simulink model "XFLUID02_reference"  (R2025a)
settings: Solver=ode23t  StartTime=0  StopTime=1.5  MaxStep=0.001  RelTol=1e-3  EnableMultiTasking=on
model workspace (MAT data in the model file):
  TRP_Par : object (value not decoded)
  fault_cylinder = 2
  inlet_area_factor = 1
  output_pressure_bar = 7
  pOutMeas_data = [7; 7]
  pOutMeas_time = [0; 1.5]
  pOut_Init_WKSP = 7
  pump_speed_rpm = 958
  seal_leak_fraction = 0
  speed_step_fraction = 0.08
  speed_step_time = 0.72
symbols that are objects in the model workspace (value not decoded): TRP_Par
undefined symbols (not defined in the file): Plunger, sm_pump_triplex_lib, smiData, X, Y, Z
libraries: sm_lib x133, fl_lib x62, nesl_utility x24, SimscapeFluids_lib x15, simulink x10, ee_lib x2
(part 7 of 7)

== system XFLUID02_reference/Pump/Plunger 3/Seal Leak/Tune ==
  Fixed Orifice : SimscapeFluids_lib/Isothermal Liquid/Valves & Orifices/Orifices/Orifice (IL)  orifice_type=1  constant_orifice_spec=fluids.isothermal_liquid.valves_orifices.orifices.enum.constant_orifice_spec.area  variable_orifice_spec=fluids.isothermal_liquid.valves_orifices.orifices.enum.orifice_spec.linear  orifice_area_constant=leak_cyl_area_WKSP m^2  p_diff_TLU_constant=[-4, -3, -2, -1, -.5, 0, .5, 1, 2, 3, 4] MPa  vol_flow_TLU_constant=[-2.44, -2.12, -1.68, -1.22, -.84, 0, .85, 1.21, 1.7, 2.09, 2.41] .* 1e-3 m^3/s  S_min=0 m  del_S=5e-3 m  open_orientation=fluids.isothermal_liquid.valves_orifices.orifices.enum.orifice_orientation.positive  area_max=1e-4 m^2  area_leak=1e-10 m^2  S_TLU=[0, .002, .004, .007, .017] m  orifice_area_TLU=[1e-09, 2.0352e-07, 4.0736e-05, .00011438, .00034356] m^2  area=inf m^2  Cd=0.7  Re_c=150  smoothing_factor=0.01  pressure_recovery=false  S_vol_flow_TLU=[0, .002, .004, .007, .017] m  p_diff_TLU=[.3, .5, .7] MPa  vol_flow_TLU=1e-3 * [1.7e-05, 2e-05, 2.6e-05; .0035, .0045, .0053; .7, .9, 1.06; 1.96, 2.5, 3; 6, 7.7, 9.13] m^3/s
      settings: LibrarySourceBlock=sh_lib/Orifices/Fixed Orifice  InternalSimscapePortConfiguration="{\"Bottom\":[],\"Left\":[{\"id\":\"A\",\"label\":\"A\",\"type\":\"foundation.isothermal_liquid.isothermal_liquid\"}],\"Right\":[{\"id\":\"B\",\"label\":\"B\",\"type\":\"foundation.isothermal_liquid.isothermal_liquid\"}],\"Top\":[]}"
  Hydraulic Reference : fl_lib/Isothermal Liquid/Elements/Reservoir (IL)  reservoir_type=foundation.enum.constant_controlled.constant  pressure_spec=foundation.enum.pressure_spec.atmospheric  reservoir_pressure=0.101325 MPa
      settings: LibrarySourceBlock=fl_lib/Hydraulic/Hydraulic Elements/Hydraulic Reference
  A : PMIOPort  Side=Left
  connections:
  Fixed Orifice/RConn1 -- Hydraulic Reference/LConn1
  Fixed Orifice/LConn1 -- A/RConn1

== system XFLUID02_reference/Pump/Plunger 3/Valve Visual/Off ==
  qi : Inport
  qo : Inport  Port=2
  Reference Frame : sm_lib/Frames and Transforms/Reference Frame
  Terminator : Terminator
  Terminator1 : Terminator
  W : PMIOPort  Side=Right
  wires:
  qi/1 -> Terminator1/1
  qo/1 -> Terminator/1
  connections:
  Reference Frame/RConn1 -- W/RConn1

== system XFLUID02_reference/Pump/Plunger 3/Valve Visual/On ==
  qi : Inport
  qo : Inport  Port=2
  Check Ball In : sm_lib/Body Elements/Spherical Solid  SphereRadius=chkv_vis_rad_in  SphereRadiusUnits=m  ExportEntireGeometry=off  InertiaType=CalculateFromGeometry  BasedOnType=Density  Density=1000  DensityUnits=kg/m^3  Mass=1  MassUnits=kg  CenterOfMass=[0 0 0]  CenterOfMassUnits=m  MomentsOfInertia=[1 1 1]  MomentsOfInertiaUnits=kg*m^2  ProductsOfInertia=[1 1 1]  ProductsOfInertiaUnits=kg*m^2  GraphicType=FromGeometry  MarkerShape=Sphere  MarkerSize=10  GraphicVisPropType=SimpleVisualProperties  GraphicDiffuseColor=chkv_vis_clr_in  GraphicOpacity=1.0  GraphicSpecularColor=[0.5 0.5 0.5 1.0]  GraphicAmbientColor=[0.15 0.15 0.15 1.0]  GraphicEmissiveColor=[0.0 0.0 0.0 1.0]  GraphicShininess=75  DoExposeReferenceFrame=on  SerializedFrames=<Frames/>
  Check Ball Out : sm_lib/Body Elements/Spherical Solid  SphereRadius=chkv_vis_rad_out  SphereRadiusUnits=m  ExportEntireGeometry=off  InertiaType=CalculateFromGeometry  BasedOnType=Density  Density=1000  DensityUnits=kg/m^3  Mass=1  MassUnits=kg  CenterOfMass=[0 0 0]  CenterOfMassUnits=m  MomentsOfInertia=[1 1 1]  MomentsOfInertiaUnits=kg*m^2  ProductsOfInertia=[1 1 1]  ProductsOfInertiaUnits=kg*m^2  GraphicType=FromGeometry  MarkerShape=Sphere  MarkerSize=10  GraphicVisPropType=SimpleVisualProperties  GraphicDiffuseColor=chkv_vis_clr_out  GraphicOpacity=1.0  GraphicSpecularColor=[0.5 0.5 0.5 1.0]  GraphicAmbientColor=[0.15 0.15 0.15 1.0]  GraphicEmissiveColor=[0.0 0.0 0.0 1.0]  GraphicShininess=75  DoExposeReferenceFrame=on  SerializedFrames=<Frames/>
  Gain : Gain  Gain=-1
  Prismatic Check Ball In : sm_lib/Joints/Prismatic Joint  JointMode=Normal  CompositeWrenchDir=FollowerOnBase  CompositeWrenchFrame=BaseFrame  SenseConstraintForce=off  SenseConstraintTorque=off  SenseTotalForce=off  SenseTotalTorque=off  PositionTargetSpecify=off  PositionTargetPriority=High  PositionTargetValue=0  PositionTargetValueUnits=m  VelocityTargetSpecify=off  VelocityTargetPriority=High  VelocityTargetValue=0  VelocityTargetValueUnits=m/s  EquilibriumPosition=0  EquilibriumPositionUnits=m  SpringStiffness=0  SpringStiffnessUnits=N/m  DampingCoefficient=0  DampingCoefficientUnits=N/(m/s)  LowerLimitSpecify=off  LowerLimitBound=-1  LowerLimitBoundUnits=m  LowerLimitStiffness=1e6  LowerLimitStiffnessUnits=N/m  LowerLimitDamping=1e3  LowerLimitDampingUnits=N/(m/s)  LowerLimitTransitionRegionWidth=1e-4  LowerLimitTransitionRegionWidthUnits=m  UpperLimitSpecify=off  UpperLimitBound=1  UpperLimitBoundUnits=m  UpperLimitStiffness=1e6  UpperLimitStiffnessUnits=N/m  UpperLimitDamping=1e3  UpperLimitDampingUnits=N/(m/s)  UpperLimitTransitionRegionWidth=1e-4  UpperLimitTransitionRegionWidthUnits=m  TorqueActuationMode=ComputedTorque  MotionActuationMode=InputMotion  SensePosition=off  SenseVelocity=off  SenseAcceleration=off  SenseTorqueForce=off  SenseLowerLimitTorqueForce=off  SenseUpperLimitTorqueForce=off
  Prismatic Check Ball Out : sm_lib/Joints/Prismatic Joint  JointMode=Normal  CompositeWrenchDir=FollowerOnBase  CompositeWrenchFrame=BaseFrame  SenseConstraintForce=off  SenseConstraintTorque=off  SenseTotalForce=off  SenseTotalTorque=off  PositionTargetSpecify=off  PositionTargetPriority=High  PositionTargetValue=0  PositionTargetValueUnits=m  VelocityTargetSpecify=off  VelocityTargetPriority=High  VelocityTargetValue=0  VelocityTargetValueUnits=m/s  EquilibriumPosition=0  EquilibriumPositionUnits=m  SpringStiffness=0  SpringStiffnessUnits=N/m  DampingCoefficient=0  DampingCoefficientUnits=N/(m/s)  LowerLimitSpecify=off  LowerLimitBound=-1  LowerLimitBoundUnits=m  LowerLimitStiffness=1e6  LowerLimitStiffnessUnits=N/m  LowerLimitDamping=1e3  LowerLimitDampingUnits=N/(m/s)  LowerLimitTransitionRegionWidth=1e-4  LowerLimitTransitionRegionWidthUnits=m  UpperLimitSpecify=off  UpperLimitBound=1  UpperLimitBoundUnits=m  UpperLimitStiffness=1e6  UpperLimitStiffnessUnits=N/m  UpperLimitDamping=1e3  UpperLimitDampingUnits=N/(m/s)  UpperLimitTransitionRegionWidth=1e-4  UpperLimitTransitionRegionWidthUnits=m  TorqueActuationMode=ComputedTorque  MotionActuationMode=InputMotion  SensePosition=off  SenseVelocity=off  SenseAcceleration=off  SenseTorqueForce=off  SenseLowerLimitTorqueForce=off  SenseUpperLimitTorqueForce=off
  Simulink-PS Converter : nesl_utility/Simulink-PS Converter  PhysicalDomain=network_engine_domain  SubClassName=ps_input  LeftPortType=input  RightPortType=output  PseudoPeriodic=off  Frequencies=[]  NoiseDistribution=none  NoiseParameters=[]  Unit=m  AffineConversion=off  FilteringAndDerivatives=filter  SimscapeFilterOrder=2  InputFilterTimeConstant=0.005  UdotUserProvided=0
  Simulink-PS Converter1 : nesl_utility/Simulink-PS Converter  PhysicalDomain=network_engine_domain  SubClassName=ps_input  LeftPortType=input  RightPortType=output  PseudoPeriodic=off  Frequencies=[]  NoiseDistribution=none  NoiseParameters=[]  Unit=m  AffineConversion=off  FilteringAndDerivatives=filter  SimscapeFilterOrder=2  InputFilterTimeConstant=0.005  UdotUserProvided=0
  Transform Inlet : sm_lib/Frames and Transforms/Rigid Transform  RotationMethod=None  FollAlignAxisA=+X  BaseAlignAxisA=+Y  FollAlignAxisB=+Y  BaseAlignAxisB=+Z  RotationStandardAxis=+Z  RotationAngle=0.0  RotationAngleUnits=deg  RotationArbitraryAxis=[0 0 1]  RotationSequenceAxes=FollowerAxes  RotationSequence=XYX  RotationSequenceAngles=[0 0 0]  RotationSequenceAnglesUnits=deg  RotationMatrix=[1 0 0; 0 1 0; 0 0 1]  Quaternion=[1 0 0 0]  TranslationMethod=Cartesian  TranslationCartesianOffset=[0 -0.04 -0.055-0.005]  TranslationCartesianOffsetUnits=m  TranslationStandardAxis=+Z  TranslationStandardOffset=0  TranslationStandardOffsetUnits=m  TranslationROffset=0  TranslationROffsetUnits=m  TranslationThetaOffset=0  TranslationThetaOffsetUnits=deg  TranslationZOffset=0  TranslationZOffsetUnits=m
  Transform Outlet : sm_lib/Frames and Transforms/Rigid Transform  RotationMethod=StandardAxis  FollAlignAxisA=+X  BaseAlignAxisA=+Y  FollAlignAxisB=+Y  BaseAlignAxisB=+Z  RotationStandardAxis=-X  RotationAngle=90  RotationAngleUnits=deg  RotationArbitraryAxis=[0 0 1]  RotationSequenceAxes=FollowerAxes  RotationSequence=XYX  RotationSequenceAngles=[0 0 0]  RotationSequenceAnglesUnits=deg  RotationMatrix=[1 0 0; 0 1 0; 0 0 1]  Quaternion=[1 0 0 0]  TranslationMethod=Cartesian  TranslationCartesianOffset=[0 0.020 -0.063]  TranslationCartesianOffsetUnits=m  TranslationStandardAxis=+Z  TranslationStandardOffset=0  TranslationStandardOffsetUnits=m  TranslationROffset=0  TranslationROffsetUnits=m  TranslationThetaOffset=0  TranslationThetaOffsetUnits=deg  TranslationZOffset=0  TranslationZOffsetUnits=m
  W : PMIOPort  Side=Right
  wires:
  Gain/1 -> Simulink-PS Converter/1
  qo/1 -> Simulink-PS Converter1/1
  qi/1 -> Gain/1
  connections:
  Simulink-PS Converter1/RConn1 -- Prismatic Check Ball Out/LConn2
  Prismatic Check Ball Out/RConn1 -- Check Ball Out/RConn1
  Prismatic Check Ball Out/LConn1 -- Transform Outlet/RConn1
  Simulink-PS Converter/RConn1 -- Prismatic Check Ball In/LConn2
  Transform Inlet/RConn1 -- Prismatic Check Ball In/LConn1
  W/RConn1 -- Transform Inlet/LConn1 -- Transform Outlet/LConn1
  Prismatic Check Ball In/RConn1 -- Check Ball In/RConn1

== system XFLUID02_reference/Driver/Driver/Motor/Windings/Enable if rotor angle 0-240 Deg ==
  Ang : Inport
  Constant2 : Constant  Value=360
  Interval Test : simulink/Logic and Bit Operations/Interval Test  IntervalClosedRight=on  uplimit=240  IntervalClosedLeft=on  lowlimit=0  OutDataTypeStr=uint8
      settings: AttributesFormatString=%<lowlimit><angle<%<uplimit>
  Math Function : Math  Operator=rem  SignedPower=on
  En : Outport  VectorParamsAs1DForOutWhenUnconnected=off
  wires:
  Constant2/1 -> Math Function/2
  Math Function/1 -> Interval Test/1
  Interval Test/1 -> En/1
  Ang/1 -> Math Function/1

== matlab function XFLUID02_reference/Diagnostics/Diagnostics/On/FFT and Classification ==
  data: pArray input; faultState output; enablePred input; cmdSpeed input; hmiVec output
function [faultState,hmiVec] = faultClassifier(pArray,enablePred,cmdSpeed)

% Initialize Predicted Machine State
faultState = int8(0);
hmiVec = [1 0 0 0];

% Sampling Parameters
Np = 1000;
Dt = 0.001;
numFreqPeaks = 5;

% Initialize Prediction Algorithm Input
predIn = NaN(1,2*numFreqPeaks+1);

pAvg = mean(pArray);

% Load Trained Machine Learning Algorithm
pumpPredict = loadLearnerForCoder('sm_pump_triplex_fault_detect_algo');

if enablePred
    
    % Compute FFT of Accumulated Data
    [freq,mag] = getFFTData(Np,pArray,Dt);
    
    % Normalize FFT Results
    freqFaultSpd = freq*60/(2*pi)/(cmdSpeed*3);

    % Detect FFT Peak Frequencies
    [pks,loc] = findpeaks(mag,'MinPeakProminence',0.5e-3);

    % Center FFT Peak Frequencies around Primary Machine Frequency
    normSpd = abs(freqFaultSpd(loc)-1);
    [sortFreq,sortIdx] = sort(normSpd);
    sortMag = pks(sortIdx);

    % Only Update Detected Peaks
    if length(sortMag) <= numFreqPeaks
        numFreq = length(sortMag);
    else
        numFreq = numFreqPeaks;
    end
    
    % Construct Input Array for Machine Learning Algorithm
    for i = 1:numFreq
        predIn(2*(i-1)+1) = sortFreq(i);
        predIn(2*i) = sortMag(i);
        predIn(i+1) = sortMag(i);
    end
    predIn(2*numFreqPeaks+1) = pAvg;
    
    % Predict Machine State using Classification Algorithm
    faultState = predict(pumpPredict,predIn);
    
    % Flag Machine Vector for HMI Indicators
    if faultState == 3 || faultState == 4 || faultState == 5
        hmiVec(2) = 1;  hmiVec(1) = 0;
    end
    if faultState == 1 || faultState == 2 || faultState == 4
        hmiVec(3) = 1;  hmiVec(1) = 0;
    end
    if faultState == 2 || faultState == 5 || faultState == 7
        hmiVec(4) = 1;  hmiVec(1) = 0;
    end
    
else
    % 
    faultState = int8(0);
    hmiVec = [0 0 0 0];
end
end

function [freq, mag] = getFFTData(np,yout,dt)
% Code to calculate frequency response data
%
% Copyright 2017 The MathWorks, Inc.

% % Compute fft
yout_intp = yout(:).*hamming(np);
f = fft(yout_intp)/np;
f2 = f(1:(np/2)+1);
w = (0:np/2)/np*(2*pi/dt);
P = abs(f2);
ind = 20 < w & w < 525; % Between 20 & 525 radians/sec
freq = w(ind)';
mag = P(ind);
end

== matlab function XFLUID02_reference/Diagnostics/Diagnostics/On/Collect Data ==
  data: pOut input; pArray output
function pArray  = dataAccum(pOut)

persistent pOutArray

Np = 1000;

if isempty(pOutArray)
    pOutArray = zeros(Np,1);
end

pOutArray = [pOut; pOutArray(1:Np-1)];
pArray = pOutArray;
end
